simulink model "wind_gen"  (R2024b)
settings: Solver=VariableStepAuto  StartTime=0.0  StopTime=0.005  RelTol=1e-3
libraries: spsGroundLib x1, spsPermanentMagnetSynchronousMachineLib x1, eePowerMeasurement x1, spsThreePhaseSeriesRLCBranchLib x1, spsThreePhaseVIMeasurementLib x1, sps_lib x1
settings Model: Creator=Aswin  LastModifiedBy=Mahesh

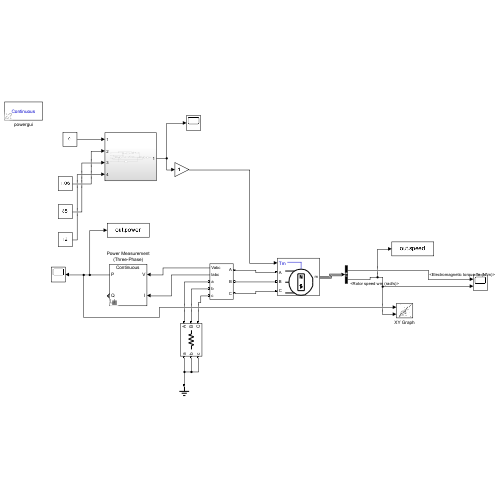
[thumbnail: Simulink's stored preview of the top-level diagram]
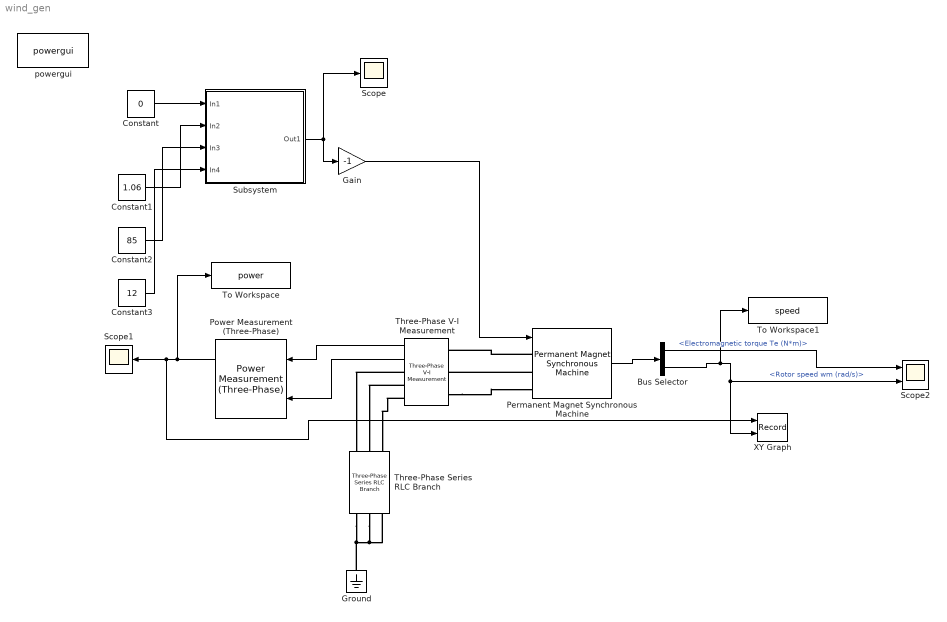
== system wind_gen ==
  Bus Selector : BusSelector  OutputSignals=Electromagnetic torque Te (N*m),Rotor speed wm (rad/s)
  Constant : Constant  Value=0
  Constant1 : Constant  Value=1.06
  Constant2 : Constant  Value=85
  Constant3 : Constant  Value=12
  Gain : Gain  Gain=-1
  Ground : spsGroundLib/Ground  LConnTagsString=a
  Permanent Magnet Synchronous Machine : spsPermanentMagnetSynchronousMachineLib/Permanent Magnet Synchronous Machine  NbPhases=3  FluxDistribution=Sinusoidal  RotorType=Round  MechanicalLoad=Torque Tm  PresetModel=No  ShowDetailedParameters=on  MeasurementBus=off  Resistance=0.0485  Inductance=8.5e-3  dqInductances=[8.5e-3,8.5e-3]  La=0.000395  MachineConstant=Flux linkage established by magnets (V.s)  Flux=0.1194  VoltageCst=86.6271  TorqueCst=0.7164  Flat=120  Mechanical=[0.0027 0.0004924 4 0]  PolePairs=4  InitialConditions=[0,0, 0,0]  InitialConditions5ph=[0 0 0 0 0 0]  RefAngle=90 degrees behind phase A axis (modified Park)  IterativeDiscreteModel=Trapezoidal non iterative  TsBlock=-1  TsPowergui=0
  Power Measurement (Three-Phase) : eePowerMeasurement/Power Measurement (Three-Phase)  LabelModeActiveChoice=Continuous  F=60  K=[0 1 2 3]  Seq=Positive  Ts=0
  Scope : Scope
  Scope1 : Scope
  Scope2 : Scope  NumInputPorts=2
  Subsystem : Subsystem
  Three-Phase Series RLC Branch : spsThreePhaseSeriesRLCBranchLib/Three-Phase Series RLC Branch  LConnTagsString=A|B|C  RConnTagsString=A|B|C  BranchType=R  Resistance=10000  Inductance=1e-3  Capacitance=1e-6  Measurements=None
  Three-Phase V-I Measurement : spsThreePhaseVIMeasurementLib/Three-Phase V-I Measurement  VoltageMeasurement=phase-to-ground  SetLabelV=off  LabelV=Vabc  Vpu=off  VpuLL=off  CurrentMeasurement=yes  SetLabelI=off  LabelI=Iabc  Ipu=off  Pbase=100e6  Vbase=500e3  OutputType=Complex  PhasorSimulation=off  PSBequivalent=0
  To Workspace : ToWorkspace  VariableName=power  SaveFormat=Timeseries  SampleTime=-1
  To Workspace1 : ToWorkspace  VariableName=speed  SaveFormat=Timeseries  SampleTime=-1
  XY Graph : Record  FileSettingsInternal="{\"entries\":[{\"content\":{\"excelSettings\":{\"content\":{},\"type\":\"Streamout.ExcelSettings\"}},\"type\":\"Streamout.FileSettingStorage\",\"uuid\":\"\"}],\"packageUris\":[\"http:\\/\\/schema.mathworks.com\\/mf0\\/streamout_blocks\\/R2020a\"],\"version\":\"1.0\"}"  Layout=[1 1]  SignalsInternal="{\"entries\":[{\"content\":{\"signals\":[{\"content\":{\"blockPath\":[],\"dimensions\":[4],\"domain\":\"\",\"hasChildren\":true,\"lineColor\":\"#77ac30\",\"lineWidth\":2,\"port\":1,\"sid\":[\"\"],\"signalID\":1,\"signalName\":\"Power Measurement\\n(Three-Phase):1\"},\"type\":\"RecordBlkView.Signal\",\"uuid\":\"\"},{\"content\":{\"blockPath\":[],\"channel\":[1],\"dimensions\":[4],\"domain\":\"\",\"lineColor\":\"#d95319\",\"lineWidth\":2,\"parentID\":1,\"port\":1,\"sid\":[\"\"],\"signalID\":2,\"signalName\":\"Power Measurement\\n(Three-Phase):1\"},\"type\":\"RecordBlkView.Signal\",\"uuid\":\"\"},{\"content\":{\"blockPath\":[],\"dimensions\":[1],\"domain\":\"\",\"lineColor\":\"#139fff\",\"plots\":[ 1 ],\"port\":2,\"sid\":[\"\"],\"signalID\":3,\"signalName\":\"<Rotor speed wm (rad\\/s)>\"},\"type\":\"RecordBlkView.Signal\",\"uuid\":\"\"},{\"content\":{\"blockPath\":[],\"channel\":[2],\"dimensions\":[4],\"domain\":\"\",\"lineColor\":\"#a2142f\",\"lineWidth\":2,\"parentID\":1,\"port\":1,\"sid\":[\"\"],\"signalID\":4,\"signalName\":\"Power Measurement\\n(Three-Phase):1\"},\"type\":\"RecordBlkView.Signal\",\"uuid\":\"\"},{\"content\":{\"blockPath\":[],\"channel\":[3],\"dimensions\":[4],\"domain\":\"\",\"lineColor\":\"#139fff\",\"lineWidth\":2,\"parentID\":1,\"port\":1,\"sid\":[\"\"],\"signalID\":5,\"signalName\":\"Power Measurement\\n(Three-Phase):1\"},\"type\":\"RecordBlkView.Signal\",\"uuid\":\"\"},{\"content\":{\"blockPath\":[],\"channel\":[4],\"dimensions\":[4],\"domain\":\"\",\"lineColor\":\"#ff6929\",\"lineWidth\":2,\"parentID\":1,\"plots\":[ 1 ],\"port\":1,\"sid\":[\"\"],\"signalID\":6,\"signalName\":\"Power Measurement\\n(Three-Phase):1\"},\"type\":\"RecordBlkView.Signal\",\"uuid\":\"\"}]},\"type\":\"RecordBlkView.InputSignals\",\"uuid\":\"\"}],\"packageUris\":[\"http:\\/\\/schema.mathworks.com\\/mf0\\/streamout_blocks\\/R2020a\"],\"version\":\"1.0\"}"  VisualizationBindings="{\"xyplotplugin\":{\"info\":[{\"series\":[{\"bindingParametersList\":[{\"parameter\":\"X-Axis\",\"signalID\":3,\"signalName\":\"<Rotor speed wm (rad\\/s)>\"},{\"parameter\":\"Y-Axis\",\"signalID\":6,\"signalName\":\"Power Measurement\\n(Three-Phase):1(4)\"}],\"seriesID\":0}],\"subplotID\":1}]}}"  CompatibilityTag=XY
  powergui : sps_lib/powergui  Priority=1  SimulationMode=Continuous  SampleTime=50e-6  frequency=60  Iterations=50  frequencyindice=0  Pbase=100e6  ErrMax=1e-4  UnitsV=kV  UnitsW=MW  buscounter=0  FunctionMessages=off  echomessages=off  EnableUseOfTLC=off  CurrentSourceSwitches=off  DisableSnubberDevices=off  DisableRonSwitches=off  DisableVfSwitches=off  DisplayEquations=off  AutomaticDiscreteSolvers=off  SolverType=Tustin/Backward Euler (TBE)  Interpol=off  ExternalGateDelay=off  methode=off  Ts=100  x0status=blocks  SPID=on  SwTol=0  HookPort=off  NonlinearTolerance=1e-4  nMaxIteration=100  ContinueOnMaxIteration=off  RestoreLinks=warning  ResistiveCurrentMeasurement=off  Frange=[0:2:500]  Ylog=off  Xlog=on  ShowGrid=off  save=off  variable=ZData  structure=0  ZoomFFT=off  StartTime=0.0  cycles=1  DisplayStyle=1  fundamental=60  FreqAxis=off  MaxFrequency=1000  frequencyindicesteady=1  RmsSteady=1  display=off
  wires:
  Constant/1 -> Subsystem/1(In1)
  Constant1/1 -> Subsystem/2(In2)
  Constant2/1 -> Subsystem/3(In3)
  Constant3/1 -> Subsystem/4(In4)
  Subsystem/1(Out1) -> Gain/1, Scope/1
  Power Measurement (Three-Phase)/1 -> To Workspace/1, XY Graph/1, Scope1/1
  Three-Phase V-I Measurement/1 -> Power Measurement (Three-Phase)/1
  Three-Phase V-I Measurement/2 -> Power Measurement (Three-Phase)/2
  Gain/1 -> Permanent Magnet Synchronous Machine/1
  Permanent Magnet Synchronous Machine/1 -> Bus Selector/1
  Bus Selector/1 -> Scope2/1  "<Electromagnetic torque Te (N*m)>"
  Bus Selector/2 -> To Workspace1/1, XY Graph/2, Scope2/2  "<Rotor speed wm (rad/s)>"
  connections:
  Three-Phase V-I Measurement/RConn1 -- Three-Phase Series RLC Branch/LConn1
  Three-Phase V-I Measurement/RConn2 -- Three-Phase Series RLC Branch/LConn2
  Three-Phase V-I Measurement/RConn3 -- Three-Phase Series RLC Branch/LConn3
  Permanent Magnet Synchronous Machine/LConn1 -- Three-Phase V-I Measurement/LConn1
  Permanent Magnet Synchronous Machine/LConn2 -- Three-Phase V-I Measurement/LConn2
  Three-Phase V-I Measurement/LConn3 -- Permanent Magnet Synchronous Machine/LConn3
  Ground/LConn1 -- Three-Phase Series RLC Branch/RConn1 -- Three-Phase Series RLC Branch/RConn2 -- Three-Phase Series RLC Branch/RConn3

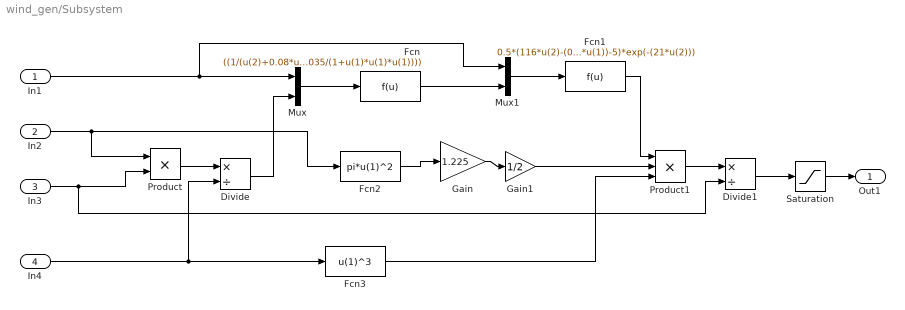
== system wind_gen/Subsystem ==
  In1 : Inport
  In2 : Inport  Port=2
  In3 : Inport  Port=3
  In4 : Inport  Port=4
  Divide : Product  Inputs=*/
  Divide1 : Product  Inputs=*/
  Fcn : Fcn  Expr=((1/(u(2)+0.08*u(1)))-(0.035/(1+u(1)*u(1)*u(1))))
  Fcn1 : Fcn  Expr=0.5*(116*u(2)-(0.4*u(1))-5)*exp(-(21*u(2)))
  Fcn2 : Fcn  Expr=pi*u(1)^2
  Fcn3 : Fcn  Expr=u(1)^3
  Gain : Gain  Gain=1.225
  Gain1 : Gain  Gain=1/2
  Mux : Mux  Inputs=2
  Mux1 : Mux  Inputs=2
  Product : Product
  Product1 : Product  Inputs=3
  Saturation : Saturate  UpperLimit=inf  LowerLimit=1e-2
  Out1 : Outport
  wires:
  In3/1 -> Divide1/2, Product/2
  Product/1 -> Divide/1
  In1/1 -> Mux1/1, Mux/1
  Divide/1 -> Mux/2
  Mux/1 -> Fcn/1
  Fcn/1 -> Mux1/2
  Mux1/1 -> Fcn1/1
  In2/1 -> Product/1, Fcn2/1
  In4/1 -> Divide/2, Fcn3/1
  Fcn2/1 -> Gain/1
  Gain/1 -> Gain1/1
  Gain1/1 -> Product1/2
  Fcn1/1 -> Product1/1
  Fcn3/1 -> Product1/3
  Product1/1 -> Divide1/1
  Divide1/1 -> Saturation/1
  Saturation/1 -> Out1/1
